simulink model "DC5_closed_loop"  (R2020a)
settings: Solver=FixedStepAuto  StartTime=0.0  StopTime=inf  RelTol=1e-3  EnableMultiTasking=on
PreLoadFcn:
  | load motorResponse
  | Ts = 0.1;
values from neighbouring files (symbols this model uses):
  PWMcmdMono = [-1 -0.9 -0.85 -0.75 -0.7 -0.6 -0.55 -0.5 -0.45 -0.4 -0.35 -0.3 ... (32 elements, 32x1)]    [motorResponse.mat]
  speedMono = [-305 -300 -295 -290 -285 -275 -265 -255 -245 -230 -210 -180 ... (32 elements, 32x1)]    [motorResponse.mat]
libraries: mkrmotorcarrierlib x2
settings Model: SimulationMode=external  SILPILModeSetting=veronly  ExtModeTrigDuration=2  Creator=bnewman  LastModifiedBy=mmarathe
settings DataIOCC: ReturnWorkspaceOutputs=off
settings OptimizationCC: PassReuseOutputArgsThreshold=0  MaxStackSize=64
settings DebuggingCC: ParameterTunabilityLossMsg=error  ArithmeticOperatorsInVariantConditions=warning
settings HardwareCC: ProdBitPerPointer=32  ProdBitPerSizeT=32  ProdBitPerPtrDiffT=32  ProdLargestAtomicInteger=Long  ProdLargestAtomicFloat=Double  ProdWordSize=32  ProdHWDeviceType=ARM Compatible->ARM Cortex
settings SFSimCC: SimUseLocalCustomCode=off  MATLABDynamicMemAlloc=off  CustomCodeUndefinedFunction=UseInterfaceOnly
settings RTWCC: SystemTargetFile=ert.tlc  HardwareBoard=Arduino Nano 33 IoT  TLCOptions=-aInlineSetEventsForThisBaseRateFcn=TLC_FALSE -aSuppressMultiTaskScheduler=TLC_FALSE -aRateBasedStepFcn=1  TemplateMakefile=ert_default_tmf  GenerateReport=on  RTWUseLocalCustomCode=off  Toolchain=Arduino ARM  BuildConfiguration=Faster Runs  LaunchReport=on
settings CodeAppCC: ForceParamTrailComments=on  OperatorAnnotations=on
settings ERTTargetCC: ERTCustomFileBanners=off  SupportContinuousTime=on  SupportNonInlinedSFcns=on  RemoveResetFunc=off  SupportVariableSizeSignals=on  ModelStepFunctionPrototypeControlCompliant=off  ExtModeStaticAllocSize=8192

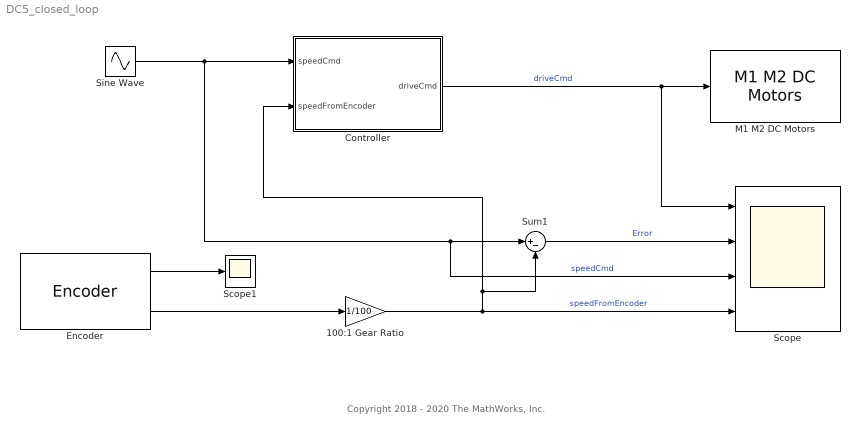
== system DC5_closed_loop ==
  note: Copyright 2018 - 2020 The MathWorks, Inc.
  100:1 Gear Ratio : Gain  Gain=1/100
  Controller : Subsystem
  Encoder : mkrmotorcarrierlib/Encoder  SlaveAddress=uint8( hex2dec( '66' ) )  blockPlatform=ARDUINO  Encoder=1  ShowSpeed=on  ResetOption=on  SampleTime=0.1
      settings: SourceProductName=Simulink Support for Arduino MKR Motor Carrier
  M1 M2 DC Motors : mkrmotorcarrierlib/M1 M2 DC Motors  SlaveAddress=uint8( hex2dec( '66' ) )  blockPlatform=ARDUINO  MotorNumber=M1  MotorCarrierPWMFreq=100
      settings: SourceProductBaseCode=ARDUINO
  Scope : Scope  NumInputPorts=4
  Scope1 : Scope
  Sine Wave : Sin  Amplitude=200  SampleTime=Ts
  Sum1 : Sum  Inputs=|+-
  wires:
  Encoder/2 -> 100:1 Gear Ratio/1
  100:1 Gear Ratio/1 -> Controller/2(speedFromEncoder), Sum1/2, Scope/4  "speedFromEncoder"
  Sum1/1 -> Scope/2  "Error"
  Encoder/1 -> Scope1/1
  Sine Wave/1 -> Scope/3, Sum1/1, Controller/1(speedCmd)  "speedCmd"
  Controller/1(driveCmd) -> M1 M2 DC Motors/1, Scope/1  "driveCmd"

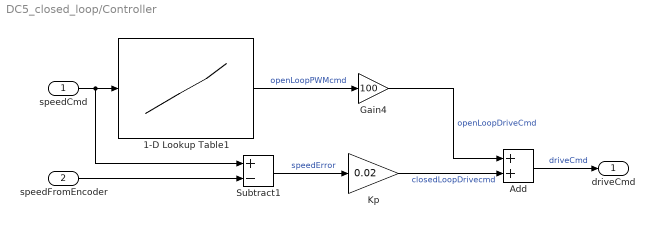
== system DC5_closed_loop/Controller ==
  speedCmd : Inport
  speedFromEncoder : Inport  Port=2
  1-D Lookup Table1 : Lookup_n-D  NumberOfTableDimensions=1  BreakpointsForDimension1=speedMono  Table=PWMcmdMono  InternalRulePriority=Speed  RndMeth=Simplest  InputSameDT=on
  Add : Sum
  Gain4 : Gain  Gain=100
  Kp : Gain  Gain=0.02
  Subtract1 : Sum  Inputs=+-
  driveCmd : Outport  VectorParamsAs1DForOutWhenUnconnected=off
  wires:
  Gain4/1 -> Add/1  "openLoopDriveCmd"
  Subtract1/1 -> Kp/1  "speedError"
  Kp/1 -> Add/2  "closedLoopDrivecmd"
  1-D Lookup Table1/1 -> Gain4/1  "openLoopPWMcmd"
  Add/1 -> driveCmd/1  "driveCmd"
  speedFromEncoder/1 -> Subtract1/2
  speedCmd/1 -> Subtract1/1, 1-D Lookup Table1/1
